simulink model "PV_CC_Ppv0p1_Pcc0p8"  (R2023b)
settings: Solver=FixedStepAuto  StartTime=0.0  StopTime=1.5  RelTol=1e-3
undefined symbols (not defined in the file or in its folder): delta_E, delta_Ppq, delta_theta_deg, enable_breaker, Lg, Rg, Sn_ccGFM, Sn_pvGFL, Tf, Ts, Vn, wQSEMvcc
libraries: spsSequenceAnalyzerLib x2, spsThreePhaseParallelRLCLoadLib x2, GFL_Lib x1, GFM_Lib x1, Source_Lib x1, spsLoadFlowBusLib x1, spsPower3phInstantaneousLib x1, spsThreePhaseSeriesRLCBranchLib x1, spsThreePhaseVIMeasurementLib x1, spsThreePhaseBreakerLib x1, VSC_Lib x1, spspowerguiLib x1
settings Model: Creator=pcstudentgele11  LastModifiedBy=pcstudentgele11

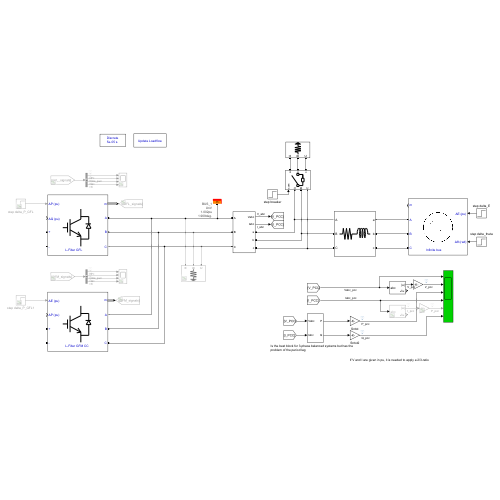
[thumbnail: Simulink's stored preview of the top-level diagram]
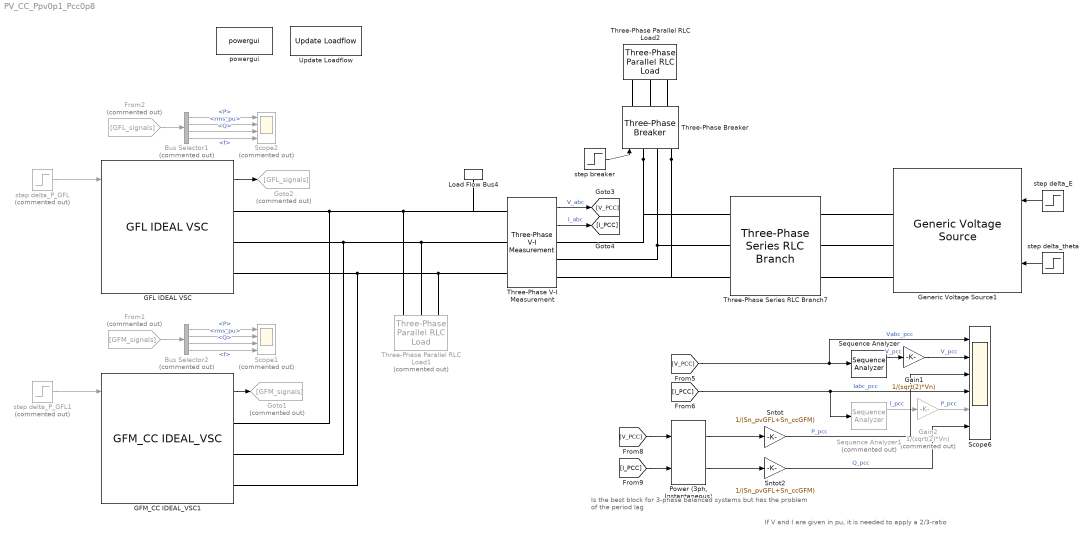
== system PV_CC_Ppv0p1_Pcc0p8 ==
  note: Is the best block for 3-phase balanced systems but has the problem of the period lag
  note: If V and I are given in pu, it is needed to apply a 2/3-ratio
  Bus Selector1 : BusSelector  Commented=on  OutputSignals=P,Vg.rms_pu,Q,f
  Bus Selector2 : BusSelector  Commented=on  OutputSignals=P,Vg.rms_pu,Q,f
  From1 : From  Commented=on  GotoTag=GFM_signals
  From2 : From  Commented=on  GotoTag=GFL_signals
  GFL IDEAL VSC : GFL_Lib/GFL IDEAL VSC  fn=fn  Sn=Sn_pvGFL  Pn=Sn_pvGFL  Udcn=Vdc  Output_Delay=Delaypv  Un1=Vnvsc  Un2=Un  m=1  Rt_pu=0.005  Lt_pu=0.15  Lm_pu=500  Rm_pu=500  DC_Link=Perfect DC Source  H_DC=inf  H_DC_sav=inf  wn_PLL=wpllpv  zeta_PLL=1  QV=Voltage Control  w_P=wppv  w_V=wvpv  w_LPF=30  wn_i=wipv  zeta_i=1  Kffi=on  Filtre_FF=on  w_ff=wffpv  Imax=1  Iqmax=0.3  K_FRT=0  Advanced=on  LFpopup=PQ  P0=Ppv  Q0=-3.0358e-17  V0=1.0023  Theta0=1.9086
      settings: SourceProductName=VSC4SPS
  GFM_CC IDEAL_VSC1 : GFM_Lib/GFM_CC IDEAL_VSC  fn=fn  Sn=Sn_ccGFM  Pn=Sn_ccGFM  Udcn=Vdc  Output_Delay=Delaycc  Un1=Vnvsc  Un2=Un  Rt_pu=0.005  Lt_pu=0.15  Lm_pu=500  Rm_pu=500  DC_Link=Perfect DC Source  H_DC=inf  H_DC_sav=inf  wn_PLL=50  zeta_PLL=1  Val_Freq_Support=on  R_percent=8  dLc_pu=0  Rv=0.09  W_TVR=60  I_max_pu=1.2  Tr_I_max=10  Tau_fCC=1/wQSEMvcc  wn_CC=wicc  Kffi=on  Filtre_FF=off  w_ff=wffcc  Advanced=on  gainpopup=With Inertia  wn_Inertia_Less=5/(2*pi)  Param_Inertia=PI  H_GFo=Hcc  zeta_GFo=ksicc  LFpopup=PQ  P0=Pcc  Q0=-0.014366  V0=1.0023  Theta0=1.9086
      settings: SourceProductName=VSC4SPS
  Gain1 : Gain  Gain=1/(sqrt(2)*Vn)
  Gain2 : Gain  Commented=on  Gain=1/(sqrt(2)*Vn)
  Generic Voltage Source1 : Source_Lib/Generic Voltage Source  SourceNature_str=INFINITE  fn=fn  Sn=Sng  Un=Un  H_s=5  DroopOnOff=on  R_percent=4  TN=1  TD=2  Time_Step=Ts  LFpopup=Swing  P0=-0.099667  Q0=0.0047552  V0=1  Theta0=0
      settings: SourceProductName=VSC4SPS
  Goto1 : Goto  Commented=on  GotoTag=GFM_signals
  Goto2 : Goto  Commented=on  GotoTag=GFL_signals
  Load Flow Bus4 : spsLoadFlowBusLib/Load Flow Bus  LConnTagsString=a  Phases=single  Connectors=on one side  ID=BUS_1  Vbase=Un  Vref=1  Vangle=0  VLF=1.002  VLFb=1  VLFc=1  angleLF=1.909  angleLFb=0  angleLFc=0
  "Power (3ph, Instantaneous)" : spsPower3phInstantaneousLib/Power (3ph, Instantaneous)
  Scope1 : Scope  Commented=on  NumInputPorts=4
  Scope2 : Scope  Commented=on  NumInputPorts=4
  Scope6 : Scope  NumInputPorts=6
  Sequence Analyzer : spsSequenceAnalyzerLib/Sequence Analyzer  Freq=50  n=1  seq=Positive  InInit=[sqrt(2)*Vn, 0.953500]  Ts=0
  Sequence Analyzer1 : spsSequenceAnalyzerLib/Sequence Analyzer  Commented=on  Freq=50  n=1  seq=Positive  InInit=[0.5, 0]  Ts=0
  Sntot : Gain  Gain=1/(Sn_pvGFL+Sn_ccGFM)
  Sntot2 : Gain  Gain=1/(Sn_pvGFL+Sn_ccGFM)
  Three-Phase Parallel RLC Load1 : spsThreePhaseParallelRLCLoadLib/Three-Phase Parallel RLC Load  Commented=on  LConnTagsString=A|B|C  Configuration=Y (grounded)  NominalVoltage=Un  Vabc=[1e3 1e3 1e3]  Vabcp=[1e3 1e3 1e3]  NominalFrequency=fn  UnbalancedPower=off  ActivePower=5  InductivePower=0  CapacitivePower=0  Pabc=[10e3 9e3 11e3]  QLabc=[100 90 110]  QCabc=[100 90 110]  Pabcp=[10e3 9e3 11e3]  QLabcp=[100 90 110]  QCabcp=[100 90 110]  Measurements=None  LoadType=constant Z
  Three-Phase Parallel RLC Load2 : spsThreePhaseParallelRLCLoadLib/Three-Phase Parallel RLC Load  LConnTagsString=A|B|C  Configuration=Y (grounded)  NominalVoltage=Un  Vabc=[1e3 1e3 1e3]  Vabcp=[1e3 1e3 1e3]  NominalFrequency=fn  UnbalancedPower=off  ActivePower=P_fault  InductivePower=Q_fault  CapacitivePower=0  Pabc=[10e3 9e3 11e3]  QLabc=[100 90 110]  QCabc=[100 90 110]  Pabcp=[10e3 9e3 11e3]  QLabcp=[100 90 110]  QCabcp=[100 90 110]  Measurements=None  LoadType=constant Z
  Three-Phase Series RLC Branch7 : spsThreePhaseSeriesRLCBranchLib/Three-Phase Series RLC Branch  LConnTagsString=A|B|C  RConnTagsString=A|B|C  BranchType=RL  Resistance=Rg  Inductance=Lg  Capacitance=1e-6  Measurements=None
  Three-Phase V-I Measurement : spsThreePhaseVIMeasurementLib/Three-Phase V-I Measurement  VoltageMeasurement=phase-to-ground  SetLabelV=off  LabelV=Vabc  Vpu=off  VpuLL=off  CurrentMeasurement=yes  SetLabelI=off  LabelI=Iabc  Ipu=off  Pbase=Sn_pvGFL+Sn_ccGFM  Vbase=Vn  OutputType=Complex  PhasorSimulation=off  PSBequivalent=0
  Three-Phase Breaker : spsThreePhaseBreakerLib/Three-Phase Breaker  InitialState=open  SwitchA=on  SwitchB=on  SwitchC=on  SwitchTimes=t_breaker  External=on  BreakerResistance=0.01  SnubberResistance=1e6  SnubberCapacitance=inf  Measurements=None
  Update Loadflow : VSC_Lib/Update Loadflow  ShowInLibBrowser=on
      settings: SourceProductName=VSC4SPS
  powergui : spspowerguiLib/powergui  Priority=1  SimulationMode=Discrete  SampleTime=Ts  frequency=60  Iterations=50  frequencyindice=50  Pbase=100000  ErrMax=1e-6  UnitsV=kV  UnitsW=MW  buscounter=14  FunctionMessages=off  echomessages=off  EnableUseOfTLC=off  CurrentSourceSwitches=off  DisableSnubberDevices=off  DisableRonSwitches=off  DisableVfSwitches=off  DisplayEquations=off  AutomaticDiscreteSolvers=off  SolverType=Tustin/Backward Euler (TBE)  Interpol=off  ExternalGateDelay=off  methode=off  Ts=100  x0status=blocks  SPID=on  SwTol=0  HookPort=off  NonlinearTolerance=1e-4  nMaxIteration=100  ContinueOnMaxIteration=off  RestoreLinks=warning  ResistiveCurrentMeasurement=off  Frange=[0:2:500]  Ylog=off  Xlog=on  ShowGrid=off  save=off  variable=ZData  structure=0  ZoomFFT=off  StartTime=0.0  cycles=1  DisplayStyle=1  fundamental=60  FreqAxis=off  MaxFrequency=1000  frequencyindicesteady=1  RmsSteady=1  display=off
  step breaker : Step  Time=Tf  After=enable_breaker  SampleTime=0
  step delta_E : Step  Time=Tf  After=delta_E  SampleTime=0
  step delta_P_GFL : Step  Commented=on  Time=0.0  After=delta_Ppq  SampleTime=0
  step delta_P_GFL1 : Step  Commented=on  Time=0.0  After=delta_Ppq  SampleTime=0
  step delta_theta : Step  Time=Tf  After=delta_theta_deg*pi/180  SampleTime=0
  wires:
  Sequence Analyzer1/1 -> Gain2/1  "I_pcc"
  GFL IDEAL VSC/1 -> Goto2/1
  From2/1 -> Bus Selector1/1
  step delta_theta/1 -> Generic Voltage Source1/2
  "Power (3ph, Instantaneous)"/1 -> Sntot/1
  [I_PCC] -> "Power (3ph, Instantaneous)"/2
  step delta_E/1 -> Generic Voltage Source1/1
  Sequence Analyzer/1 -> Gain1/1  "V_pcc"
  Bus Selector1/2 -> Scope2/2  "<rms_pu>"
  Bus Selector1/3 -> Scope2/3  "<Q>"
  step breaker/1 -> Three-Phase Breaker/1
  [V_PCC] -> Scope6/1, Sequence Analyzer/1  "Vabc_pcc"
  Bus Selector1/1 -> Scope2/1  "<P>"
  "Power (3ph, Instantaneous)"/2 -> Sntot2/1
  Bus Selector1/4 -> Scope2/4  "<f>"
  [V_PCC] -> "Power (3ph, Instantaneous)"/1
  step delta_P_GFL/1 -> GFL IDEAL VSC/1
  Three-Phase V-I Measurement/2 -> [I_PCC]  "I_abc"
  Three-Phase V-I Measurement/1 -> [V_PCC]  "V_abc"
  [I_PCC] -> Scope6/4, Sequence Analyzer1/1  "Iabc_pcc"
  GFM_CC IDEAL_VSC1/1 -> Goto1/1
  Bus Selector2/1 -> Scope1/1  "<P>"
  From1/1 -> Bus Selector2/1
  Bus Selector2/2 -> Scope1/2  "<rms_pu>"
  Bus Selector2/4 -> Scope1/4  "<f>"
  Bus Selector2/3 -> Scope1/3  "<Q>"
  step delta_P_GFL1/1 -> GFM_CC IDEAL_VSC1/1
  Sntot/1 -> Scope6/3  "P_pcc"
  Sntot2/1 -> Scope6/6  "Q_pcc"
  Gain1/1 -> Scope6/2  "V_pcc"
  Gain2/1 -> Scope6/5  "P_pcc"
  connections:
  GFL IDEAL VSC/RConn2 -- GFM_CC IDEAL_VSC1/RConn2 -- Three-Phase Parallel RLC Load1/LConn2 -- Three-Phase V-I Measurement/LConn2
  Three-Phase Breaker/LConn3 -- Three-Phase Series RLC Branch7/LConn3 -- Three-Phase V-I Measurement/RConn3
  Three-Phase Breaker/LConn1 -- Three-Phase Series RLC Branch7/LConn1 -- Three-Phase V-I Measurement/RConn1
  Three-Phase Parallel RLC Load1/LConn1 -- Three-Phase V-I Measurement/LConn1 -- Load Flow Bus4/LConn1 -- GFM_CC IDEAL_VSC1/RConn1 -- GFL IDEAL VSC/RConn1
  GFL IDEAL VSC/RConn3 -- GFM_CC IDEAL_VSC1/RConn3 -- Three-Phase Parallel RLC Load1/LConn3 -- Three-Phase V-I Measurement/LConn3
  Three-Phase Breaker/LConn2 -- Three-Phase Series RLC Branch7/LConn2 -- Three-Phase V-I Measurement/RConn2
  Three-Phase Series RLC Branch7/RConn3 -- Generic Voltage Source1/RConn3
  Three-Phase Parallel RLC Load2/LConn1 -- Three-Phase Breaker/RConn1
  Three-Phase Series RLC Branch7/RConn2 -- Generic Voltage Source1/RConn2
  Three-Phase Breaker/RConn3 -- Three-Phase Parallel RLC Load2/LConn3
  Three-Phase Series RLC Branch7/RConn1 -- Generic Voltage Source1/RConn1
  Three-Phase Breaker/RConn2 -- Three-Phase Parallel RLC Load2/LConn2
